simulink model "XAERO01_reference"  (R2025a)
settings: Solver=FixedStepDiscrete  StartTime=0  StopTime=18  FixedStep=0.002  RelTol=1e-3
undefined symbols (not defined in the file): gust_factor, gust_time, payload_mass, payload_release_time, target_x, target_y, target_z, wind_heading, wind_speed
settings Model: Creator=SimuVerity Contributors  LastModifiedBy=SimuVerity Contributors

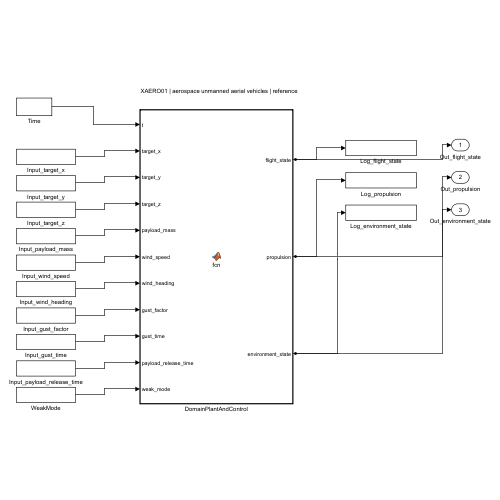
[thumbnail: Simulink's stored preview of the top-level diagram]
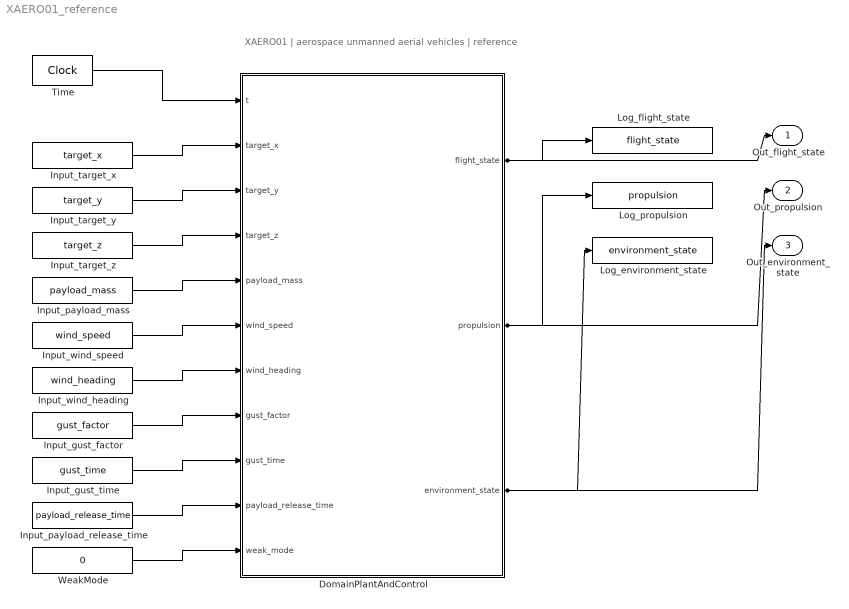
== system XAERO01_reference ==
  note: XAERO01 | aerospace unmanned aerial vehicles | reference
  DomainPlantAndControl : MATLAB Function  TreatAsAtomicUnit=on
  Input_gust_factor : Constant  Value=gust_factor
  Input_gust_time : Constant  Value=gust_time
  Input_payload_mass : Constant  Value=payload_mass
  Input_payload_release_time : Constant  Value=payload_release_time
  Input_target_x : Constant  Value=target_x
  Input_target_y : Constant  Value=target_y
  Input_target_z : Constant  Value=target_z
  Input_wind_heading : Constant  Value=wind_heading
  Input_wind_speed : Constant  Value=wind_speed
  Log_environment_state : ToWorkspace  VariableName=environment_state  SaveFormat=Timeseries  SampleTime=-1
  Log_flight_state : ToWorkspace  VariableName=flight_state  SaveFormat=Timeseries  SampleTime=-1
  Log_propulsion : ToWorkspace  VariableName=propulsion  SaveFormat=Timeseries  SampleTime=-1
  Time : DigitalClock  SampleTime=0.002
  WeakMode : Constant  Value=0
  Out_flight_state : Outport
  Out_propulsion : Outport  Port=2
  Out_environment_state : Outport  Port=3
  wires:
  Time/1 -> DomainPlantAndControl/1(t)
  Input_target_x/1 -> DomainPlantAndControl/2(target_x)
  Input_target_y/1 -> DomainPlantAndControl/3(target_y)
  Input_target_z/1 -> DomainPlantAndControl/4(target_z)
  Input_payload_mass/1 -> DomainPlantAndControl/5(payload_mass)
  Input_wind_speed/1 -> DomainPlantAndControl/6(wind_speed)
  Input_wind_heading/1 -> DomainPlantAndControl/7(wind_heading)
  Input_gust_factor/1 -> DomainPlantAndControl/8(gust_factor)
  Input_gust_time/1 -> DomainPlantAndControl/9(gust_time)
  Input_payload_release_time/1 -> DomainPlantAndControl/10(payload_release_time)
  WeakMode/1 -> DomainPlantAndControl/11(weak_mode)
  DomainPlantAndControl/1(flight_state) -> Log_flight_state/1, Out_flight_state/1
  DomainPlantAndControl/2(propulsion) -> Log_propulsion/1, Out_propulsion/1
  DomainPlantAndControl/3(environment_state) -> Log_environment_state/1, Out_environment_state/1

== matlab function XAERO01_reference/DomainPlantAndControl ==
  data: t input; flight_state output; target_x input; target_y input; target_z input; payload_mass input; wind_speed input; wind_heading input; gust_factor input; gust_time input; payload_release_time input; weak_mode input; propulsion output; environment_state output
function [flight_state,propulsion,environment_state] = fcn(t,target_x,target_y,target_z,payload_mass,wind_speed,wind_heading,gust_factor,gust_time,payload_release_time,weak_mode)
%#codegen
persistent pos vel ang rate thrust intPos energy
dt=.002; g=9.81; baseMass=3.2; arm=.32; kyaw=.018; I=[.092,.098,.165];
if isempty(pos) || t<.5*dt
    pos=zeros(1,3); vel=zeros(1,3); ang=zeros(1,3); rate=zeros(1,3);
    thrust=((baseMass+payload_mass)*g/4)*ones(1,4); intPos=zeros(1,3); energy=180;
end
attached=payload_mass*double(t<payload_release_time); mass=baseMass+attached;
head=wind_heading*pi/180; wind=[wind_speed*cos(head),wind_speed*sin(head),0];
gust=double(t>=gust_time && t<gust_time+1.2);
wind=wind+gust_factor*wind_speed*gust*[-sin(head),cos(head),.15];
ramp=min(max((t-.5)/3.0,0),1); ref=ramp*[target_x,target_y,target_z];
e=ref-pos; intPos=min(max(intPos+e*dt,-14),14);
vdes=min(max(.80*e,-4.2),4.2);
drag=.075*(wind-vel).*abs(wind-vel);
if weak_mode<.5
    aCmd=2.40*(vdes-vel); Fcmd=mass*aCmd-drag; tiltLim=.62;
    rollDes=min(max(-Fcmd(2)/(mass*g),-tiltLim),tiltLim);
    pitchDes=min(max(Fcmd(1)/(mass*g),-tiltLim),tiltLim);
    thrustDes=min(max((mass*(g+aCmd(3))-drag(3))/max(cos(rollDes)*cos(pitchDes),.72),0),76);
    moment=[4.8*(rollDes-ang(1))-1.65*rate(1),4.8*(pitchDes-ang(2))-1.65*rate(2),2.2*(-ang(3))-1.05*rate(3)];
else
    aCmd=.72*(vdes-vel); rollDes=min(max(-aCmd(2)/g,-.18),.18); pitchDes=min(max(aCmd(1)/g,-.18),.18);
    nominalMass=baseMass+1.1; thrustDes=min(max(nominalMass*(g+aCmd(3)),0),70);
    moment=[2.6*(rollDes-ang(1))-.85*rate(1),2.6*(pitchDes-ang(2))-.85*rate(2),1.0*(-ang(3))-.45*rate(3)];
end
base=thrustDes/4; dR=moment(1)/(4*arm); dP=moment(2)/(4*arm); dY=moment(3)/(4*kyaw);
desired=[base-dR-dP+dY,base+dR-dP-dY,base-dR+dP-dY,base+dR+dP+dY];
desired=min(max(desired,0),20); thrust=thrust+dt*(desired-thrust)/.045;
roll=ang(1); pitch=ang(2); yaw=ang(3); T=sum(thrust);
thrustWorld=[T*(sin(pitch)*cos(yaw)+sin(roll)*sin(yaw)),T*(sin(pitch)*sin(yaw)-sin(roll)*cos(yaw)),T*cos(roll)*cos(pitch)];
acc=(thrustWorld+drag)/mass-[0,0,g]; vel=vel+dt*acc; pos=pos+dt*vel;
actualMoment=[arm*((thrust(2)+thrust(4))-(thrust(1)+thrust(3))),arm*((thrust(3)+thrust(4))-(thrust(1)+thrust(2))),kyaw*(thrust(1)-thrust(2)-thrust(3)+thrust(4))];
gyro=[(I(3)-I(2))*rate(2)*rate(3),(I(1)-I(3))*rate(1)*rate(3),(I(2)-I(1))*rate(1)*rate(2)];
dRate=(actualMoment-gyro-[.12,.12,.08].*rate)./I; rate=rate+dt*dRate;
ct=cos(ang(2)); ct=max(ct,.15); eulerRate=[rate(1)+rate(2)*sin(ang(1))*tan(ang(2))+rate(3)*cos(ang(1))*tan(ang(2)),rate(2)*cos(ang(1))-rate(3)*sin(ang(1)),rate(2)*sin(ang(1))/ct+rate(3)*cos(ang(1))/ct];
ang=ang+dt*eulerRate;
rotorSpeed=235*sqrt(max(thrust,0)); power=6*sum(max(thrust,0).^1.5); energy=max(energy-dt*power/3600,0);
flight_state=[pos,vel,ang,rate]; propulsion=[thrust,rotorSpeed,power,energy]; environment_state=[wind,attached];
end
